simulink model "InvertedPendulum_ClosedLoop_Reference"  (R2023a)
settings: Solver=ode4  StartTime=0.0  StopTime=5  FixedStep=0.001  RelTol=1e-3
settings Model: Creator=Fasih  LastModifiedBy=Fasih

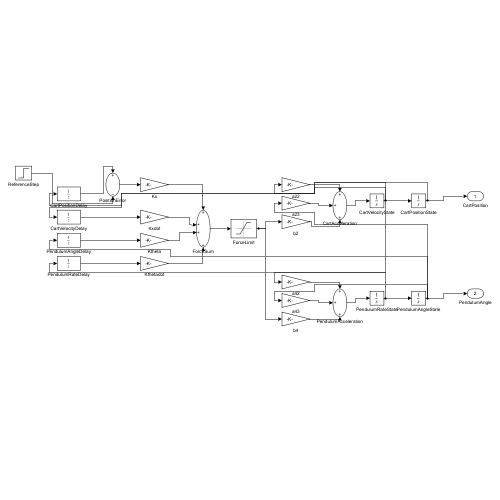
[thumbnail: Simulink's stored preview of the top-level diagram]
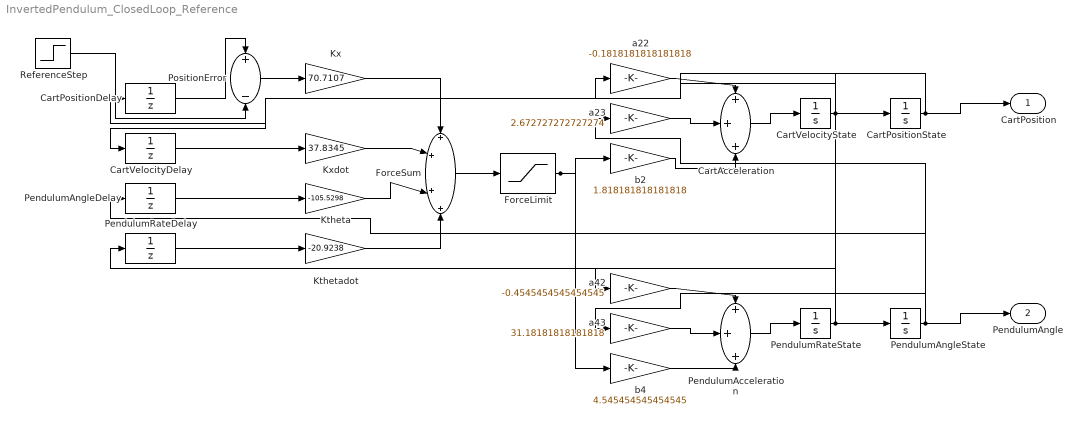
== system InvertedPendulum_ClosedLoop_Reference ==
  CartAcceleration : Sum  Inputs=+++
  CartPositionDelay : UnitDelay  SampleTime=0.001  HasFrameUpgradeWarning=on
  CartPositionState : Integrator
  CartVelocityDelay : UnitDelay  SampleTime=0.001  HasFrameUpgradeWarning=on
  CartVelocityState : Integrator
  ForceLimit : Saturate  UpperLimit=10  LowerLimit=-10
  ForceSum : Sum  Inputs=++++
  Ktheta : Gain  Gain=-105.5298
  Kthetadot : Gain  Gain=-20.9238
  Kx : Gain  Gain=70.7107
  Kxdot : Gain  Gain=37.8345
  PendulumAcceleration : Sum  Inputs=+++
  PendulumAngleDelay : UnitDelay  InitialCondition=0.08  SampleTime=0.001  HasFrameUpgradeWarning=on
  PendulumAngleState : Integrator  InitialCondition=0.08
  PendulumRateDelay : UnitDelay  SampleTime=0.001  HasFrameUpgradeWarning=on
  PendulumRateState : Integrator
  PositionError : Sum  Inputs=+-
  ReferenceStep : Step  Time=0  After=0.1  SampleTime=0
  a22 : Gain  Gain=-0.1818181818181818
  a23 : Gain  Gain=2.672727272727274
  a42 : Gain  Gain=-0.4545454545454545
  a43 : Gain  Gain=31.18181818181818
  b2 : Gain  Gain=1.818181818181818
  b4 : Gain  Gain=4.545454545454545
  CartPosition : Outport
  PendulumAngle : Outport  Port=2
  wires:
  CartPositionDelay/1 -> PositionError/1
  ReferenceStep/1 -> PositionError/2
  PositionError/1 -> Kx/1
  CartVelocityDelay/1 -> Kxdot/1
  PendulumAngleDelay/1 -> Ktheta/1
  PendulumRateDelay/1 -> Kthetadot/1
  Kx/1 -> ForceSum/1
  Kxdot/1 -> ForceSum/2
  Ktheta/1 -> ForceSum/3
  Kthetadot/1 -> ForceSum/4
  ForceSum/1 -> ForceLimit/1
  CartVelocityState/1 -> a22/1, CartPositionState/1, a42/1, CartVelocityDelay/1
  PendulumAngleState/1 -> a23/1, a43/1, PendulumAngle/1, PendulumAngleDelay/1
  ForceLimit/1 -> b2/1, b4/1
  a22/1 -> CartAcceleration/1
  a23/1 -> CartAcceleration/2
  b2/1 -> CartAcceleration/3
  CartAcceleration/1 -> CartVelocityState/1
  a42/1 -> PendulumAcceleration/1
  a43/1 -> PendulumAcceleration/2
  b4/1 -> PendulumAcceleration/3
  PendulumAcceleration/1 -> PendulumRateState/1
  PendulumRateState/1 -> PendulumAngleState/1, PendulumRateDelay/1
  CartPositionState/1 -> CartPosition/1, CartPositionDelay/1
